simulink model "Solar and Wind Hybrid DC Power Supply"  (R2024a)
settings: Solver=VariableStepAuto  StartTime=0.0  StopTime=0.5  RelTol=1e-3
libraries: spsVoltageMeasurementLib x8, spsSeriesRLCBranchLib x7, spsCurrentMeasurementLib x3, spsDiodeLib x2, spsIGBTDiodeLib x2, spsGroundLib x1, spsPVArrayLib x1, spsPWMGeneratorDCDCLib x1, spsPermanentMagnetSynchronousMachineLib x1, spsUniversalBridgeLib x1, spsWindTurbineLib x1, sps_lib x1
settings Model: Creator=DELL  LastModifiedBy=hp
settings RTWCC: GPUComputeCapability=3.5

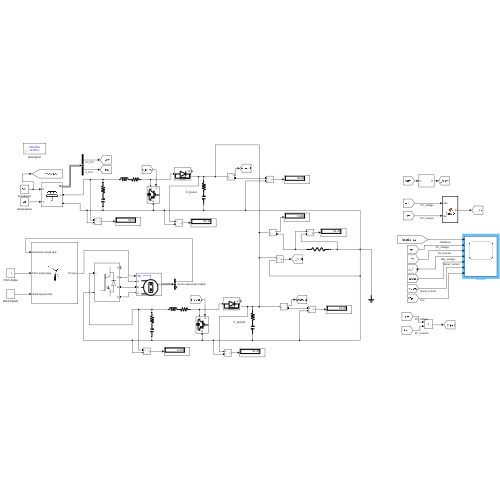
[thumbnail: Simulink's stored preview of the top-level diagram]
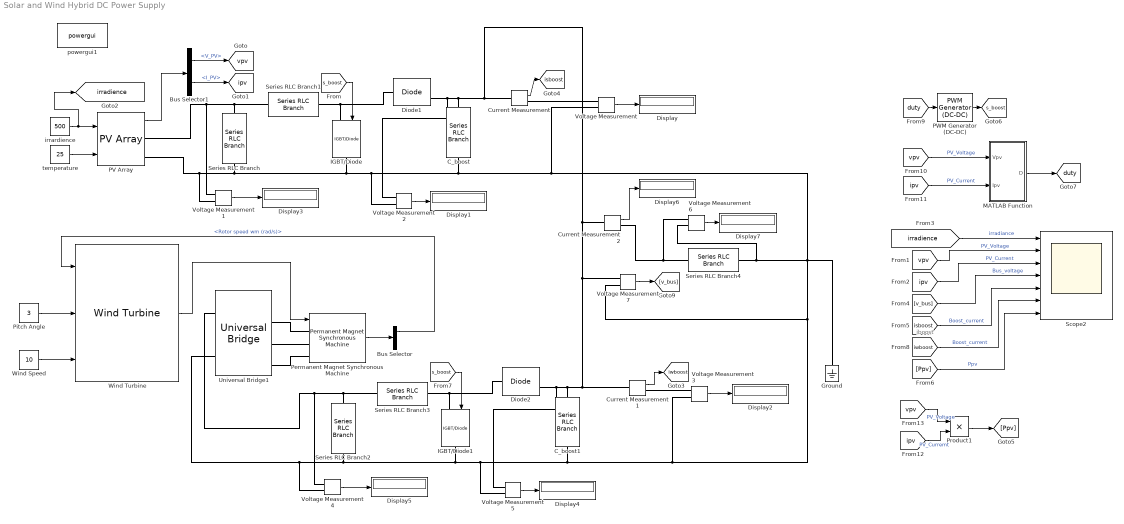
== system Solar and Wind Hybrid DC Power Supply ==
  note: iboost
  Bus Selector : BusSelector  OutputSignals=Rotor speed wm (rad/s),Rotor speed wm (rad/s)
  Bus Selector1 : BusSelector  OutputSignals=V_PV,I_PV
  C_boost : spsSeriesRLCBranchLib/Series RLC Branch  LConnTagsString=__new0  RConnTagsString=__new0  BranchType=RC  Resistance=1e-4  Inductance=1e-3  SetiL0=off  InitialCurrent=0  Capacitance=3300e-5  Setx0=off  InitialVoltage=0  Measurements=None
  C_boost1 : spsSeriesRLCBranchLib/Series RLC Branch  LConnTagsString=__new0  RConnTagsString=__new0  BranchType=RC  Resistance=1e-4  Inductance=1e-3  SetiL0=off  InitialCurrent=0  Capacitance=3300e-5  Setx0=off  InitialVoltage=0  Measurements=None
  Current Measurement : spsCurrentMeasurementLib/Current Measurement  PhasorSimulation=off  OutputType=Complex  PSBequivalent=0
  Current Measurement1 : spsCurrentMeasurementLib/Current Measurement  PhasorSimulation=off  OutputType=Complex  PSBequivalent=0
  Current Measurement2 : spsCurrentMeasurementLib/Current Measurement  PhasorSimulation=off  OutputType=Complex  PSBequivalent=0
  Diode1 : spsDiodeLib/Diode  Ron=0.001  Lon=0  Vf=0.8  IC=0  UseSnubber=0  Rs=500  Cs=250e-9  Measurements=on
  Diode2 : spsDiodeLib/Diode  Ron=0.001  Lon=0  Vf=0.8  IC=0  UseSnubber=0  Rs=500  Cs=250e-9  Measurements=on
  Display{,1..7} (8 alike) : Display
  Ground : spsGroundLib/Ground  LConnTagsString=a
  IGBT/Diode : spsIGBTDiodeLib/IGBT//Diode  Ron=1e-3  Rs=1e5  Cs=inf  Measurements=off
  IGBT/Diode1 : spsIGBTDiodeLib/IGBT//Diode  Ron=1e-3  Rs=1e5  Cs=inf  Measurements=off
  MATLAB Function : MATLAB Function  TreatAsAtomicUnit=on
  PV Array : spsPVArrayLib/PV Array  Npar=5  Nser=1  PlotType=array @ 1000 W/m2 & specified temperatures  S_vec="[ 1000  500  100 ]"  Temp_C_vec="[ 45 25  ]"  ModuleName=User-defined  PlotWhenSelected=off  Pm=213.15  Ncell=60  Voc=36.3  Isc=7.84  Vm=29  Im=7.35  beta_Voc_pc=-0.36099  alpha_Isc_pc=0.102  beta_Voc=-0.13104  alpha_Isc=0.0079968  IL=7.8654  I0=2.9273e-10  nI=0.98119  Rsh=313.0553  Rs=0.39381  RobustModel=off  RobustCellTemperature=313.3991  BAL=on  Tc=1e-6  Tfilter=5e-5
  PWM Generator (DC-DC) : spsPWMGeneratorDCDCLib/PWM Generator (DC-DC)  Fsw=5000  Ts=10e-6
  Permanent Magnet Synchronous Machine : spsPermanentMagnetSynchronousMachineLib/Permanent Magnet Synchronous Machine  NbPhases=3  FluxDistribution=Sinusoidal  RotorType=Round  MechanicalLoad=Torque Tm  PresetModel=No  ShowDetailedParameters=on  MeasurementBus=off  Resistance=0.0485  Inductance=8.5e-3  dqInductances=[8.5e-3,8.5e-3]  La=0.000395  MachineConstant=Flux linkage established by magnets (V.s)  Flux=0.1194  VoltageCst=86.6271  TorqueCst=0.7164  Flat=120  Mechanical=[0.0027 0.0004924 4 0]  PolePairs=4  InitialConditions=[0,0, 0,0]  InitialConditions5ph=[0 0 0 0 0 0]  RefAngle=90 degrees behind phase A axis (modified Park)  IterativeDiscreteModel=Trapezoidal non iterative  TsBlock=-1  TsPowergui=0
  Pitch Angle : Constant  Value=3
  Product1 : Product
  Scope2 : Scope  NumInputPorts=7
  Series RLC Branch : spsSeriesRLCBranchLib/Series RLC Branch  LConnTagsString=__new0  RConnTagsString=__new0  BranchType=RC  Resistance=1e-4  Inductance=1e-3  SetiL0=off  InitialCurrent=0  Capacitance=1000e-5  Setx0=off  InitialVoltage=0  Measurements=None
  Series RLC Branch1 : spsSeriesRLCBranchLib/Series RLC Branch  LConnTagsString=__new0  RConnTagsString=__new0  BranchType=RL  Resistance=0.1  Inductance=5e-3  SetiL0=off  InitialCurrent=0  Capacitance=1000e-5  Setx0=off  InitialVoltage=0  Measurements=None
  Series RLC Branch2 : spsSeriesRLCBranchLib/Series RLC Branch  LConnTagsString=__new0  RConnTagsString=__new0  BranchType=RC  Resistance=1e-4  Inductance=1e-3  SetiL0=off  InitialCurrent=0  Capacitance=1000e-5  Setx0=off  InitialVoltage=0  Measurements=None
  Series RLC Branch3 : spsSeriesRLCBranchLib/Series RLC Branch  LConnTagsString=__new0  RConnTagsString=__new0  BranchType=RL  Resistance=0.1  Inductance=5e-3  SetiL0=off  InitialCurrent=0  Capacitance=1000e-5  Setx0=off  InitialVoltage=0  Measurements=None
  Series RLC Branch4 : spsSeriesRLCBranchLib/Series RLC Branch  LConnTagsString=__new0  RConnTagsString=__new0  BranchType=R  Resistance=10  Inductance=1e-3  SetiL0=off  InitialCurrent=0  Capacitance=1e-6  Setx0=off  InitialVoltage=0  Measurements=None
  Universal Bridge1 : spsUniversalBridgeLib/Universal Bridge  Arms=3  SnubberResistance=1e5  SnubberCapacitance=inf  Device=IGBT / Diodes  Ron=1e-3  Lon=0  ForwardVoltages="[  0  0  ]"  ForwardVoltage=0  GTOparameters=[ 10e-6 , 20e-6 ]  IGBTparameters=[ 1e-6 , 2e-6 ]  Measurements=None  Measurements_2=None  converterType=Rectifier
  Voltage Measurement{,1..7} (8 alike) : spsVoltageMeasurementLib/Voltage Measurement  PhasorSimulation=off  OutputType=Complex  PSBequivalent=0
  Wind Speed : Constant  Value=10
  Wind Turbine : spsWindTurbineLib/Wind Turbine  Pnom=1.5e6  Pelec_base=1.5e6/0.9  wind_base=12  P_wind_base=0.73  speed_nom=1.2  pitch_angle=0  c1_c6="[0.51763          116          0.4            5           21     0.006795]"  cp_nom=0.48  lambda_nom=8.1
  irrardience : Constant  Value=500
  powergui1 : sps_lib/powergui  Priority=1  SimulationMode=Discrete  SampleTime=1e-05  frequency=60  Iterations=50  frequencyindice=0  Pbase=100e6  ErrMax=1e-4  UnitsV=kV  UnitsW=MW  buscounter=0  FunctionMessages=off  echomessages=off  EnableUseOfTLC=off  CurrentSourceSwitches=off  DisableSnubberDevices=off  DisableRonSwitches=off  DisableVfSwitches=off  DisplayEquations=off  AutomaticDiscreteSolvers=off  SolverType=Tustin/Backward Euler (TBE)  Interpol=off  ExternalGateDelay=off  methode=off  Ts=100  x0status=blocks  SPID=on  SwTol=0  HookPort=off  NonlinearTolerance=1e-4  nMaxIteration=100  ContinueOnMaxIteration=off  RestoreLinks=warning  ResistiveCurrentMeasurement=off  Frange=[0:2:500]  Ylog=off  Xlog=on  ShowGrid=off  save=off  variable=ZData  structure=0  ZoomFFT=off  StartTime=0.0  cycles=1  DisplayStyle=1  fundamental=60  FreqAxis=off  MaxFrequency=1000  frequencyindicesteady=1  RmsSteady=1  display=off
  temperature : Constant  Value=25
  tag scope: duty=global, ipv=global, irradience=global, isboost=global, iwboost=global, s_boost=global, vpv=global
  wires:
  Pitch Angle/1 -> Wind Turbine/2
  Wind Speed/1 -> Wind Turbine/3
  Wind Turbine/1 -> Permanent Magnet Synchronous Machine/1
  Permanent Magnet Synchronous Machine/1 -> Bus Selector/1
  Bus Selector/1 -> Wind Turbine/1  "<Rotor speed wm (rad/s)>"
  Current Measurement/1 -> [isboost]
  irrardience/1 -> [irradience], PV Array/1
  PV Array/1 -> Bus Selector1/1
  [s_boost] -> IGBT/Diode/1
  Bus Selector1/2 -> [ipv]  "<I_PV>"
  temperature/1 -> PV Array/2
  Bus Selector1/1 -> [vpv]  "<V_PV>"
  Voltage Measurement/1 -> Display/1
  Voltage Measurement2/1 -> Display1/1
  Voltage Measurement1/1 -> Display3/1
  Voltage Measurement4/1 -> Display5/1
  Voltage Measurement5/1 -> Display4/1
  [s_boost] -> IGBT/Diode1/1
  Current Measurement1/1 -> [iwboost]
  Voltage Measurement3/1 -> Display2/1
  PWM Generator (DC-DC)/1 -> [s_boost]
  MATLAB Function/1(D) -> [duty]
  [vpv] -> MATLAB Function/1(Vpv)  "PV_Voltage"
  [duty] -> PWM Generator (DC-DC)/1
  [ipv] -> MATLAB Function/2(Ipv)  "PV_Current"
  Current Measurement2/1 -> Display6/1
  Voltage Measurement6/1 -> Display7/1
  [Ppv] -> Scope2/7  "Ppv"
  [iwboost] -> Scope2/6  "Boost_current"
  [vpv] -> Product1/1  "PV_Voltage"
  [irradience] -> Scope2/1  "irradiance"
  [ipv] -> Scope2/3  "PV_Current"
  [isboost] -> Scope2/5  "Boost_current"
  [ipv] -> Product1/2  "PV_Curremt"
  [vpv] -> Scope2/2  "PV_Voltage"
  Product1/1 -> [Ppv]
  [v_bus] -> Scope2/4  "Bus_voltage"
  Voltage Measurement7/1 -> [v_bus]
  connections:
  Permanent Magnet Synchronous Machine/LConn1 -- Universal Bridge1/LConn1
  Universal Bridge1/LConn2 -- Permanent Magnet Synchronous Machine/LConn2
  Permanent Magnet Synchronous Machine/LConn3 -- Universal Bridge1/LConn3
  Series RLC Branch/LConn1 -- Voltage Measurement1/LConn1 -- PV Array/RConn1 -- Series RLC Branch1/RConn1
  IGBT/Diode/LConn1 -- Series RLC Branch1/LConn1 -- Diode1/LConn1
  Voltage Measurement/LConn1 -- Current Measurement/RConn1
  Series RLC Branch3/RConn1 -- Series RLC Branch2/LConn1 -- Universal Bridge1/RConn1 -- Voltage Measurement4/LConn1
  Voltage Measurement/LConn2 -- IGBT/Diode/RConn1 -- Voltage Measurement1/LConn2 -- PV Array/RConn2 -- Series RLC Branch/RConn1 -- Voltage Measurement2/LConn2 -- C_boost/RConn1 -- Ground/LConn1 -- Voltage Measurement6/LConn2 -- Series RLC Branch4/RConn1 -- Voltage Measurement7/LConn2 -- C_boost1/RConn1 -- Voltage Measurement5/LConn2 -- IGBT/Diode1/RConn1 -- Universal Bridge1/RConn2 -- Voltage Measurement4/LConn2 -- Series RLC Branch2/RConn1 -- Voltage Measurement3/LConn2
  Diode2/LConn1 -- IGBT/Diode1/LConn1 -- Series RLC Branch3/LConn1
  C_boost/LConn1 -- Current Measurement2/LConn1 -- Voltage Measurement7/LConn1 -- Current Measurement1/LConn1 -- Voltage Measurement5/LConn1 -- Diode2/RConn1 -- C_boost1/LConn1 -- Current Measurement/LConn1 -- Voltage Measurement2/LConn1 -- Diode1/RConn1
  Voltage Measurement3/LConn1 -- Current Measurement1/RConn1
  Voltage Measurement6/LConn1 -- Series RLC Branch4/LConn1 -- Current Measurement2/RConn1

== matlab function Solar and Wind Hybrid DC Power Supply/MATLAB Function ==
  data: Vpv input; D output; Ipv input
function D = PandO(Vpv,Ipv)

persistent Dprev Pprev Vprev

%Initialize the internal vlues for the voltage and power on the
%first pass
if isempty(Dprev)
    Dprev = 0.7;
    Vprev = 190;
    Pprev = 2000;
end

% Initialize algorithm parameters
deltaD = 125e-6;

%Calculate measured array power
Ppv = Vpv*Ipv;

% Increase or decrease duty cycle based on conditions
if (Ppv-Pprev) ~= 0
    if (Ppv-Pprev) > 0
        if (Vpv-Vprev) > 0
            D = Dprev - deltaD;
        else
            D = Dprev + deltaD;
        end
    else
        if (Vpv-Vprev) > 0
            D = Dprev + deltaD;
        else
            D = Dprev - deltaD;
        end
    end
else
    D = Dprev;
end

% Update internal values
Dprev = D;
Vprev = Vpv;
Pprev = Ppv;
